simulink model "untitled"  (R2025b)
settings: Solver=VariableStepAuto  StartTime=0.0  StopTime=5  RelTol=1e-3
libraries: simulink x6
settings Model: Creator=Matthew  LastModifiedBy=Matthew

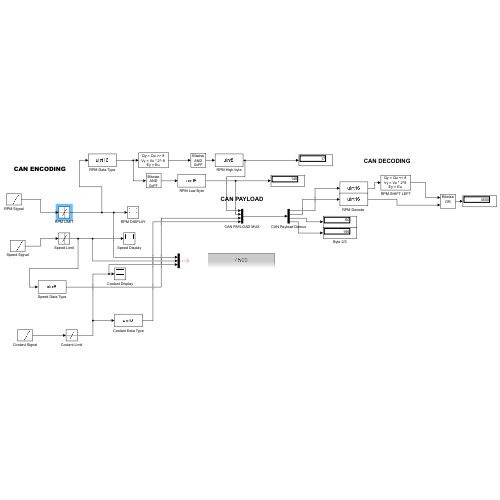
[thumbnail: Simulink's stored preview of the top-level diagram]
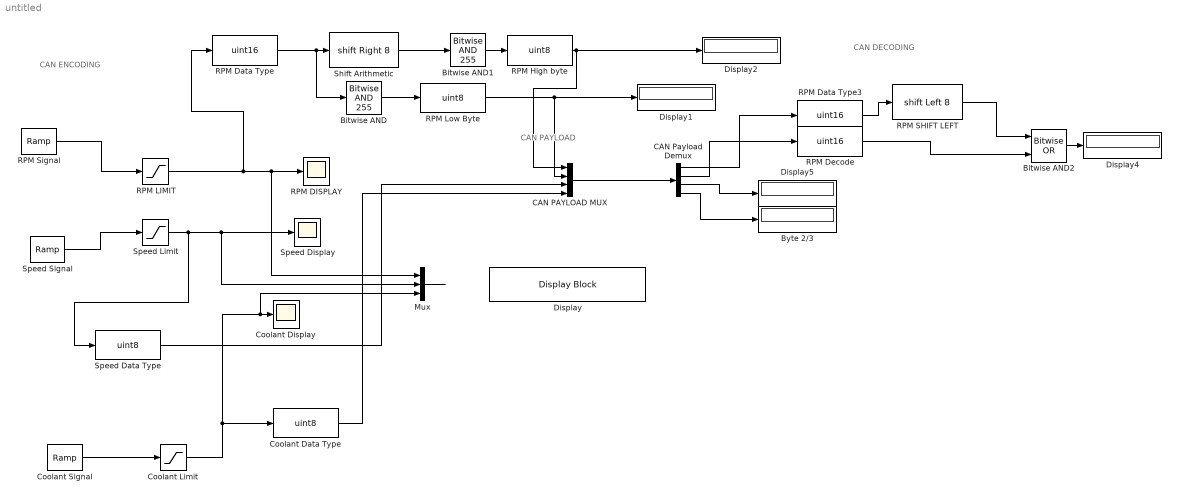
== system untitled ==
  note: CAN DECODING
  note: CAN PAYLOAD
  note: CAN ENCODING
  Bitwise AND : simulink/Logic and Bit Operations/Bitwise Operator  logicop=AND  UseBitMask=on  BitMask=255  BitMaskRealWorld=Stored Integer
      settings: LibrarySourceBlock=|
      | simulink/Quick Insert/Logic and Bit
      | Operations/Bitwise AND
  Bitwise AND1 : simulink/Logic and Bit Operations/Bitwise Operator  logicop=AND  UseBitMask=on  BitMask=255  BitMaskRealWorld=Stored Integer
      settings: LibrarySourceBlock=|
      | simulink/Quick Insert/Logic and Bit
      | Operations/Bitwise AND
  Bitwise AND2 : simulink/Logic and Bit Operations/Bitwise Operator  logicop=OR  UseBitMask=off  NumInputPorts=2  BitMask=255  BitMaskRealWorld=Stored Integer
      settings: LibrarySourceBlock=|
      | simulink/Quick Insert/Logic and Bit
      | Operations/Bitwise AND
  Byte 2/3 : Display
  CAN PAYLOAD MUX : Mux
  CAN Payload Demux : Demux
  Coolant Data Type : DataTypeConversion  OutDataTypeStr=uint8  SaturateOnIntegerOverflow=off  RndMeth=Floor  LockScale=on
  Coolant Display : Scope
      settings: ActiveDisplayYMinimum=142.94701081949898  ActiveDisplayYMaximum=374.47201081949891  DataLoggingVariableName=ScopeData2
  Coolant Limit : Saturate  UpperLimit=195  LowerLimit=170
  Coolant Signal : simulink/Sources/Ramp  slope=5  start=0  InitialOutput=170
  Display : DisplayBlock  LabelPosition=Hide  Transparency=1  GridColor=[0.502, 0.502, 0.502]
  Display{1..2,4..5} (4 alike) : Display
  Mux : Mux  Inputs=3
  RPM DISPLAY : Scope
      settings: ActiveDisplayYMinimum=582.655199749096  ActiveDisplayYMaximum=1990.6529421740311
  RPM Data Type : DataTypeConversion  OutDataTypeStr=uint16  SaturateOnIntegerOverflow=off  RndMeth=Floor  LockScale=on
  RPM Data Type3 : DataTypeConversion  OutDataTypeStr=uint16  SaturateOnIntegerOverflow=off  RndMeth=Floor  LockScale=on
  "RPM Decode " : DataTypeConversion  OutDataTypeStr=uint16  SaturateOnIntegerOverflow=off  RndMeth=Floor  LockScale=on
  RPM High byte : DataTypeConversion  OutDataTypeStr=uint8  SaturateOnIntegerOverflow=off  RndMeth=Floor  LockScale=on
  RPM LIMIT : Saturate  UpperLimit=4500  LowerLimit=900
  RPM Low Byte : DataTypeConversion  OutDataTypeStr=uint8  SaturateOnIntegerOverflow=off  RndMeth=Floor  LockScale=on
  RPM SHIFT LEFT : ArithShift  BitShiftNumber=8  BitShiftDirection=Left
  RPM Signal : simulink/Sources/Ramp  slope=800  start=0  InitialOutput=900
  Shift Arithmetic : ArithShift  BitShiftNumber=8  BitShiftDirection=Right
  Speed Data Type : DataTypeConversion  OutDataTypeStr=uint8  SaturateOnIntegerOverflow=off  RndMeth=Floor  LockScale=on
  Speed Display : Scope
      settings: ActiveDisplayYMinimum=-197.85214695929011  ActiveDisplayYMaximum=283.47169977892906
  Speed Limit : Saturate  UpperLimit=60  LowerLimit=0
  Speed Signal : simulink/Sources/Ramp  slope=12  start=0  InitialOutput=0
  wires:
  RPM LIMIT/1 -> RPM Data Type/1, RPM DISPLAY/1, Mux/1
  RPM Signal/1 -> RPM LIMIT/1
  Speed Signal/1 -> Speed Limit/1
  Speed Limit/1 -> Speed Data Type/1, Mux/2, Speed Display/1
  Coolant Signal/1 -> Coolant Limit/1
  Coolant Limit/1 -> Mux/3, Coolant Display/1, Coolant Data Type/1
  Mux/1 -> ?
  RPM Data Type/1 -> Bitwise AND/1, Shift Arithmetic/1
  Shift Arithmetic/1 -> Bitwise AND1/1
  Bitwise AND/1 -> RPM Low Byte/1
  Bitwise AND1/1 -> RPM High byte/1
  RPM Low Byte/1 -> CAN PAYLOAD MUX/2, Display1/1
  RPM High byte/1 -> CAN PAYLOAD MUX/1, Display2/1
  CAN PAYLOAD MUX/1 -> CAN Payload Demux/1
  CAN Payload Demux/3 -> Display5/1
  CAN Payload Demux/4 -> Byte 2/3/1
  Speed Data Type/1 -> CAN PAYLOAD MUX/3
  Coolant Data Type/1 -> CAN PAYLOAD MUX/4
  RPM Data Type3/1 -> RPM SHIFT LEFT/1
  Bitwise AND2/1 -> Display4/1
  CAN Payload Demux/1 -> RPM Data Type3/1
  CAN Payload Demux/2 -> "RPM Decode "/1
  RPM SHIFT LEFT/1 -> Bitwise AND2/1
  "RPM Decode "/1 -> Bitwise AND2/2
